simulink model "unit_supply_serial_rt"  (R2026b)
settings: Solver=FixedStepAuto  StopTime=inf  FixedStep=1
libraries: Lnx_ZK560103_Lib x2, simulink x1
settings Model: Creator=Administrator  LastModifiedBy=gao
settings OptimizationCC: BlockReduction=off  ReuseModelBlockBuffer=off
settings HardwareCC: ProdHWDeviceType=Intel->x86-64 (Linux 64)
settings RTWCC: SystemTargetFile=links_rtlnx_grt.tlc  TemplateMakefile=links_rtlnx_grt.tmf
settings STFCustomTargetCC: CombineOutputUpdateFcns=on  GRTInterface=off  SystemTargetFile=links_rtlnx_grt.tlc
settings GRTTargetCC: CPPClassGenCompliant=off  CompOptLevelCompliant=off  ConcurrentExecutionCompliant=off  MatFileLogging=off  ParMdlRefBuildCompliant=off  RTWCAPIParams=on  RTWCAPIRootIO=on  RTWCAPISignals=on

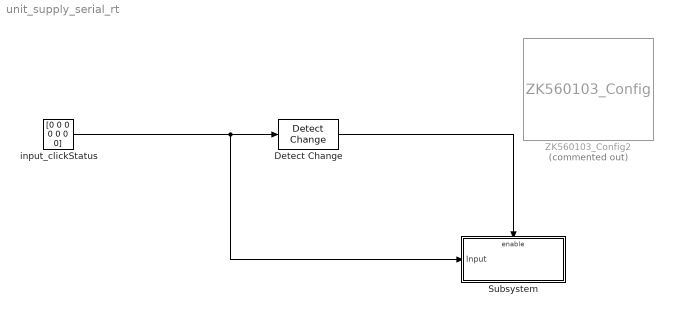
== system unit_supply_serial_rt ==
  Detect Change : simulink/Logic and Bit Operations/Detect Change  vinit=[0 0 0 0 0 0 0]  OutDataTypeStr=boolean
  Subsystem : Subsystem
  ZK560103_Config2 : Lnx_ZK560103_Lib/ZK560103_Config  Commented=on  BoardOrder=0  PortOrder=5  BaudRate=9600  Parity=0(NO PARITY)  DataBits=8  StopBits=1  mode=RS232  SampleTime=-1
      settings: SourceProductName=Links_LnxLib
  input_clickStatus : Constant  Value=[0 0 0 0 0 0 0]  VectorParams1D=off
  wires:
  input_clickStatus/1 -> Detect Change/1, Subsystem/1(Input)
  Detect Change/1 -> Subsystem/Enable

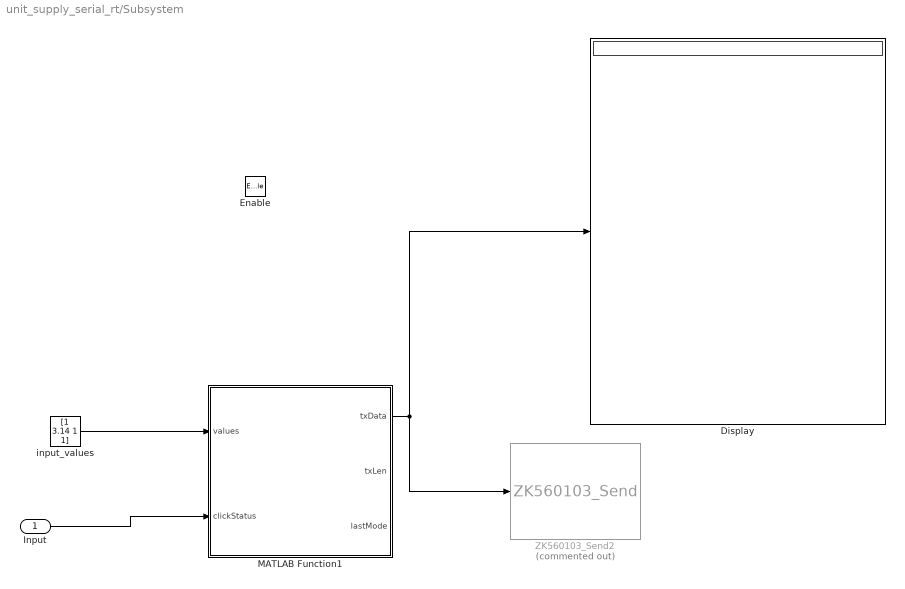
== system unit_supply_serial_rt/Subsystem ==
  Input : Inport
  Enable : EnablePort
  Display : Display
      settings: Format=hex (Stored Integer)
  MATLAB Function1 : MATLAB Function  TreatAsAtomicUnit=on
  ZK560103_Send2 : Lnx_ZK560103_Lib/ZK560103_Send  Commented=on  BoardOrder=0  PortOrder=5  sendByteType=Auto  SampleTime=-1
      settings: SourceProductName=Links_LnxLib
  input_values : Constant  Value=[1 3.14 1 1]  VectorParams1D=off
  wires:
  MATLAB Function1/1(txData) -> Display/1, ZK560103_Send2/1
  input_values/1 -> MATLAB Function1/1(values)
  Input/1 -> MATLAB Function1/2(clickStatus)

== matlab function unit_supply_serial_rt/Subsystem/MATLAB Function1 ==
  data: values input; clickStatus input; txData output; txLen output; lastMode output
function [txData, txLen, lastMode] = unit_supply_cmd_gen(values, clickStatus)
    % UDP6720系列程控电源 - SCPI命令生成函数
    %
    % values: [1x4] double 数组，分别对应 [电压设定, 电流设定, 过压保护值, 过流保护值]
    % clickStatus: [1x7] double 数组，UI控件的拨动/点击状态
    %   1: 设置电压 (发生变化即下发命令)
    %   2: 设置电流 (发生变化即下发命令)
    %   3: 输出开关 OUTPut (发生变化时下发最新状态)
    %   4: 设置过压保护值 (发生变化即下发命令)
    %   5: 设置过流保护值 (发生变化即下发命令)
    %   6: 保护功能开关 (发生变化时同时设置过压/过流保护使能)
    %   7: 测量查询按钮 (发生变化即下发命令)
    %
    % txData: uint8 命令数组 (最大 MAX_LEN 字节)
    % txLen: 命令长度
    % lastMode: 当前停留的模式 (1=CV恒压优先, 2=CC恒流优先) 用于UI指示灯显示
    %   注: UDP6720无显式模式切换，根据最后一次设定值类型判断指示

    MAX_LEN = 64;  % 电源命令稍长，适当增大缓冲区
    txData = zeros(1, MAX_LEN, 'uint8');
    txLen = 0;

    % 声明持久化变量 (相当于 Simulink 里的状态记忆)
    persistent prevClickStatus;
    persistent currentMode;

    % 初始状态赋初值 (系统刚上电时的第一拍执行)
    if isempty(prevClickStatus)
        prevClickStatus = zeros(1, 7);
    end
    if isempty(currentMode)
        currentMode = 1; % 默认停留在 1 (CV恒压模式指示)
    end

    LF = uint8(10); % 强制使用 ASCII 10 换行符 (\n) 作为SCPI结束符
    cmd = uint8([]); % 用于存放最终的字节数组

    % --- 核心逻辑：检测哪个按钮的状态发生了变化 (边缘检测) ---
    diffStatus = clickStatus - prevClickStatus;
    changedIdx = 0;
    for k = 1:7
        if abs(diffStatus(k)) > 0
            changedIdx = k;
            break;
        end
    end

    % --- 根据发生变化的按钮，组装相应的SCPI命令 ---
    if changedIdx > 0
        switch changedIdx
            case 1 % 触发了"设置电压"
                % UDP6720命令: VOLTage <value>
                currentMode = 1; % CV模式指示
                cmd = [uint8(sprintf('VOLTage %.4f', values(1))), LF];

            case 2 % 触发了"设置电流"
                % UDP6720命令: CURRent <value>
                currentMode = 2; % CC模式指示
                cmd = [uint8(sprintf('CURRent %.4f', values(2))), LF];

            case 3 % 触发了"输出开关" OUTPut
                % UDP6720命令: OUTPut ON / OUTPut OFF
                if clickStatus(3) > 0
                    cmd = [uint8('OUTPut ON'), LF];
                else
                    cmd = [uint8('OUTPut OFF'), LF];
                end

            case 4 % 触发了"设置过压保护值"
                % UDP6720命令: VOLTage:PROTection <value>
                cmd = [uint8(sprintf('VOLTage:PROTection %.4f', values(3))), LF];

            case 5 % 触发了"设置过流保护值"
                % UDP6720命令: CURRent:PROTection <value>
                cmd = [uint8(sprintf('CURRent:PROTection %.4f', values(4))), LF];

            case 6 % 触发了"保护功能开关"
                % UDP6720命令: 同时设置过压和过流保护的使能状态
                if clickStatus(6) > 0
                    cmd = [uint8('VOLTage:PROTection:STATe ON'), LF, ...
                           uint8('CURRent:PROTection:STATe ON'), LF];
                else
                    cmd = [uint8('VOLTage:PROTection:STATe OFF'), LF, ...
                           uint8('CURRent:PROTection:STATe OFF'), LF];
                end

            case 7 % 触发了"测量查询"
                % UDP6720命令: MEASure:ALL? 同时查询电压、电流、功率
                cmd = [uint8('MEASure:ALL?'), LF];
        end
    end
 
    % --- 更新记忆状态，供下一个轮询周期对比 ---
    prevClickStatus = clickStatus;
    lastMode = currentMode;

    % --- 转换为输出的底层字节 ---
    txLen = double(numel(cmd));
    if txLen > MAX_LEN
        txLen = MAX_LEN; % 防止溢出
    end
    if txLen > 0
        txData(1:txLen) = cmd(1:txLen);
    end
end
